simulink model "bengbu_model_DMPC_simple_20260715"  (R2022a)
settings: Solver=VariableStepAuto  StartTime=0.0  StopTime=84700  MaxStep=60  RelTol=1e-3
PreLoadFcn:
  | load('MPC_newmodel_20260715.mat');
InitFcn:
  | load('MPC_newmodel_20260715.mat');
StartFcn:
  | bengbu_0715_reset_workspace; bengbu_0715_export_block_params;
StopFcn:
  | bengbu_0715_schedule_finalize
undefined symbols (not defined in the file or in its folder): case3_startup_trim_prec_state, case3_startup_trim_rec_state, case3_startup_trim_reheat_state, case3_startup_trim_room_state
libraries: slpidlib x3, simulink x3, mpclib x1
settings Model: SimulationMode=accelerator  Creator=73906  LastModifiedBy=73906
settings DataIOCC: SaveOutput=off  SaveTime=off  ReturnWorkspaceOutputs=off

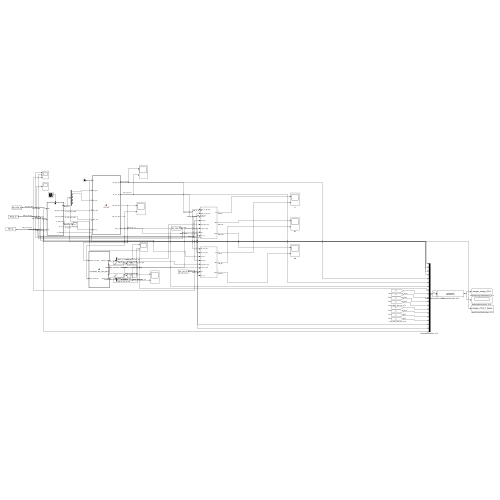
[thumbnail: Simulink's stored preview of the top-level diagram]
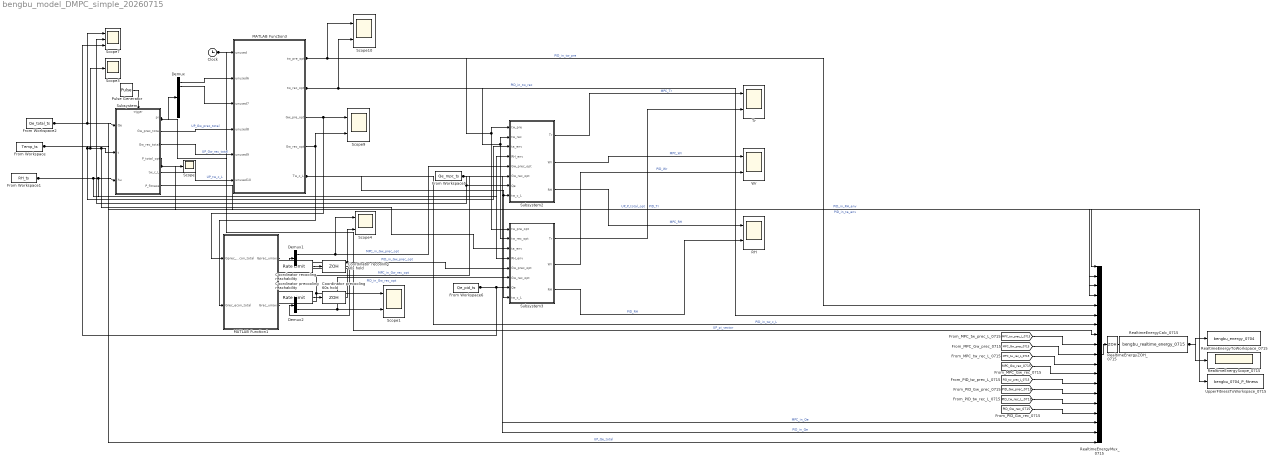
== system bengbu_model_DMPC_simple_20260715 ==
  Clock : Clock
  Coordinator precooling 60s hold : ZeroOrderHold  SampleTime=60
  Coordinator precooling reachability : RateLimiter  RisingSlewLimit=inf  FallingSlewLimit=-0.0116666666666667  InitialCondition=[4.765;4.765]
  Coordinator recooling 60s hold : ZeroOrderHold  SampleTime=60
  Coordinator recooling reachability : RateLimiter  RisingSlewLimit=inf  FallingSlewLimit=-0.02  InitialCondition=[13.2155;13.2155]
  Demux : Demux  Outputs=9
  Demux1 : Demux  Outputs=2
  Demux2 : Demux  Outputs=2
  From Workspace : FromWorkspace  VariableName=Temp_ts
  From Workspace1 : FromWorkspace  VariableName=RH_ts
  From Workspace2 : FromWorkspace  VariableName=Qe_total_ts
  From Workspace5 : FromWorkspace  VariableName=Qe_mpc_ts
  From Workspace6 : FromWorkspace  VariableName=Qe_pid_ts
  MATLAB Function1 : MATLAB Function  TreatAsAtomicUnit=on
  MATLAB Function3 : MATLAB Function  TreatAsAtomicUnit=on  SystemSampleTime=300
  Pulse Generator : DiscretePulseGenerator  PulseType=Time based  Period=3600  PulseWidth=1/360000  PhaseDelay=10
  RH : Scope  NumInputPorts=2
  RealtimeEnergyCalc_0715 : MATLABFcn  MATLABFcn=bengbu_realtime_energy_0715  OutputDimensions=31
  RealtimeEnergyMux_0715 : Mux  Inputs=19
  RealtimeEnergyScope_0715 : Scope
  RealtimeEnergyToWorkspace_0715 : ToWorkspace  VariableName=bengbu_energy_0704  SaveFormat=Timeseries  SampleTime=-1
  RealtimeEnergyZOH_0715 : ZeroOrderHold  SampleTime=300
  Scope : Scope
  Scope{1,4,9..10} (4 alike) : Scope  NumInputPorts=2
  Scope3 : Scope
  Scope7 : Scope  NumInputPorts=3
  Subsystem : Subsystem
  Subsystem2 : Subsystem
  Subsystem3 : Subsystem
  Tr : Scope  NumInputPorts=2
  UpperFitnessToWorkspace_0715 : ToWorkspace  VariableName=bengbu_0704_P_fitness  SaveFormat=Timeseries  SampleTime=-1
  Wr : Scope  NumInputPorts=2
  wires:
  Demux/2 -> MATLAB Function3/3(unused7)
  From Workspace1/1 -> Subsystem2/4(RH_env), Subsystem3/4(RH_env), Subsystem/3(hu), RealtimeEnergyMux_0715/3  "PID_in_RH_env"
  Subsystem/2(Gw_prec_total) -> MATLAB Function3/4(unused8)  "UP_Gw_prec_total"
  Subsystem/3(Gw_rec_total) -> MATLAB Function3/5(unused9)  "UP_Gw_rec_total"
  Pulse Generator/1 -> Subsystem/Trigger
  Demux/1 -> MATLAB Function3/2(unused6)
  Subsystem/1(pi) -> Demux/1, RealtimeEnergyMux_0715/8  "UP_pi_vector"
  Clock/1 -> MATLAB Function3/1(unused), RealtimeEnergyMux_0715/1
  MATLAB Function3/3(Gw_pre_opt) -> MATLAB Function1/1(Gprec_econ_total), Scope9/1
  MATLAB Function3/4(Gw_rec_opt) -> MATLAB Function1/2(Grec_econ_total), Scope9/2
  MATLAB Function3/1(tw_pre_opt) -> Subsystem2/1(tw_pre), Subsystem3/1(tw_pre_opt), Scope10/1, RealtimeEnergyMux_0715/5  "PID_in_tw_pre"
  MATLAB Function3/2(tw_rec_opt) -> Subsystem3/2(tw_rec_opt), Subsystem2/2(tw_rec), Scope10/2, RealtimeEnergyMux_0715/6  "PID_in_tw_rec"
  Subsystem2/1(Tr) -> Tr/1  "MPC_Tr"
  Demux1/1 -> Subsystem2/5(Gw_prec_opt), Scope4/1  "MPC_in_Gw_prec_opt"
  Demux1/2 -> Scope4/2, Subsystem3/5(Gw_prec_opt)  "PID_in_Gw_prec_opt"
  Demux2/1 -> Subsystem2/6(Gw_rec_opt), Scope1/1  "MPC_in_Gw_rec_opt"
  Demux2/2 -> Scope1/2, Subsystem3/6(Gw_rec_opt)  "PID_in_Gw_rec_opt"
  Subsystem3/1(Tr) -> Tr/2  "PID_Tr"
  Subsystem3/2(Wr) -> Wr/2  "PID_Wr"
  Subsystem2/2(Wr) -> Wr/1  "MPC_Wr"
  Subsystem3/3(RH) -> RH/2  "PID_RH"
  From Workspace2/1 -> Scope7/1, Subsystem/1(Qe), RealtimeEnergyMux_0715/19  "UP_Qe_total"
  From Workspace5/1 -> Scope7/2, Subsystem2/7(Qe), RealtimeEnergyMux_0715/17  "MPC_in_Qe"
  Subsystem2/3(RH) -> RH/1  "MPC_RH"
  From Workspace/1 -> Subsystem2/3(ta_env), Scope3/1, Subsystem3/3(ta_env), Subsystem/2(t), RealtimeEnergyMux_0715/2  "PID_in_ta_env"
  From Workspace6/1 -> Scope7/3, Subsystem3/7(Qe), RealtimeEnergyMux_0715/18  "PID_in_Qe"
  Subsystem/5(tw_c_L) -> MATLAB Function3/6(unused10)  "UP_tw_c_L"
  MATLAB Function3/5(Tw_c_L) -> Subsystem2/8(tw_c_L), Subsystem3/8(tw_c_L), RealtimeEnergyMux_0715/7  "PID_in_tw_c_L"
  Subsystem/4(P_total_opt) -> Scope/1, RealtimeEnergyMux_0715/4  "UP_P_total_opt"
  RealtimeEnergyMux_0715/1 -> RealtimeEnergyZOH_0715/1
  RealtimeEnergyCalc_0715/1 -> RealtimeEnergyToWorkspace_0715/1, RealtimeEnergyScope_0715/1
  [MPC_tw_prec_L_0715] -> RealtimeEnergyMux_0715/9
  [MPC_Gw_prec_0715] -> RealtimeEnergyMux_0715/10
  [MPC_tw_rec_L_0715] -> RealtimeEnergyMux_0715/11
  [MPC_Gw_rec_0715] -> RealtimeEnergyMux_0715/12
  [PID_tw_prec_L_0715] -> RealtimeEnergyMux_0715/13
  [PID_Gw_prec_0715] -> RealtimeEnergyMux_0715/14
  [PID_tw_rec_L_0715] -> RealtimeEnergyMux_0715/15
  [PID_Gw_rec_0715] -> RealtimeEnergyMux_0715/16
  RealtimeEnergyZOH_0715/1 -> RealtimeEnergyCalc_0715/1
  Subsystem/6(P_fitness) -> UpperFitnessToWorkspace_0715/1
  MATLAB Function1/1(Gprec_umax) -> Coordinator precooling reachability/1
  Coordinator precooling reachability/1 -> Coordinator precooling 60s hold/1
  Coordinator precooling 60s hold/1 -> Demux1/1
  MATLAB Function1/2(Grec_umax) -> Coordinator recooling reachability/1
  Coordinator recooling reachability/1 -> Coordinator recooling 60s hold/1
  Coordinator recooling 60s hold/1 -> Demux2/1

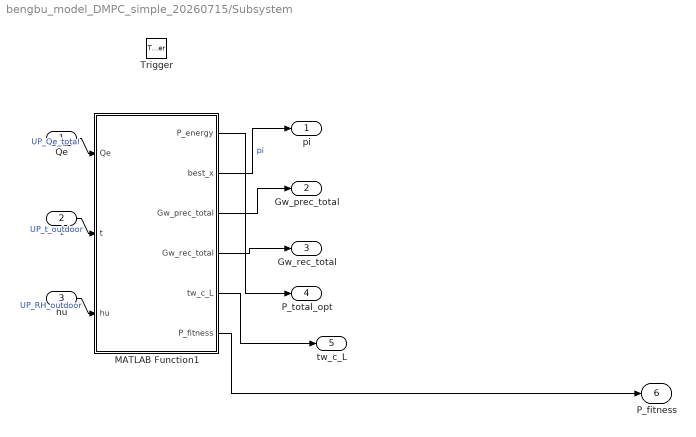
== system bengbu_model_DMPC_simple_20260715/Subsystem ==
  Qe : Inport
  t : Inport  Port=2
  hu : Inport  Port=3
  Trigger : TriggerPort  VariantControl=(inherit)  PortDimensions=1
  MATLAB Function1 : MATLAB Function  TreatAsAtomicUnit=on
  pi : Outport
  Gw_prec_total : Outport  Port=2
  Gw_rec_total : Outport  Port=3
  P_total_opt : Outport  Port=4
  tw_c_L : Outport  Port=5
  P_fitness : Outport  Port=6
  wires:
  MATLAB Function1/4(Gw_rec_total) -> Gw_rec_total/1
  MATLAB Function1/3(Gw_prec_total) -> Gw_prec_total/1
  t/1 -> MATLAB Function1/2(t)  "UP_t_outdoor"
  MATLAB Function1/2(best_x) -> pi/1  "pi"
  hu/1 -> MATLAB Function1/3(hu)  "UP_RH_outdoor"
  Qe/1 -> MATLAB Function1/1(Qe)  "UP_Qe_total"
  MATLAB Function1/1(P_energy) -> P_total_opt/1
  MATLAB Function1/5(tw_c_L) -> tw_c_L/1
  MATLAB Function1/6(P_fitness) -> P_fitness/1

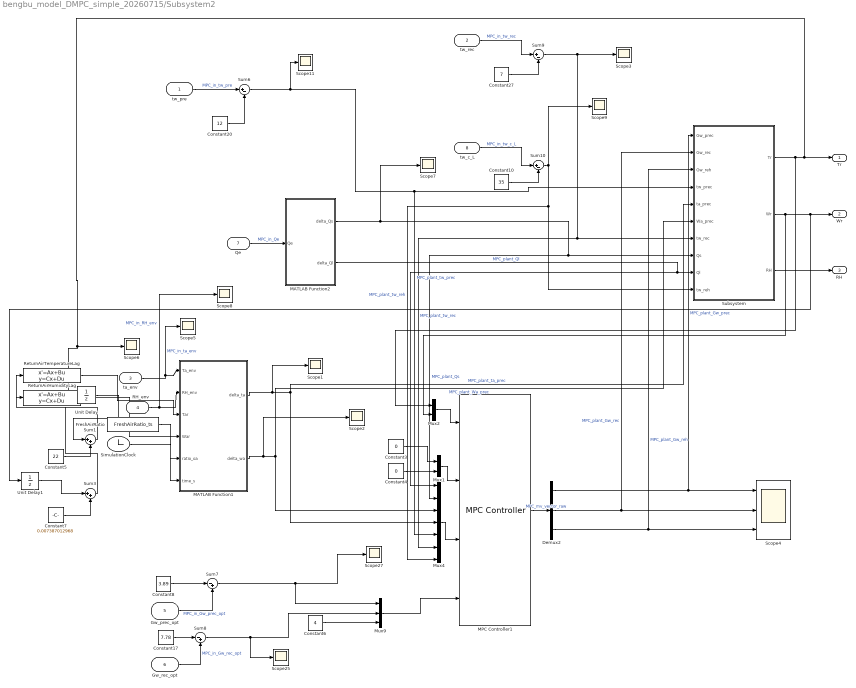
== system bengbu_model_DMPC_simple_20260715/Subsystem2 ==
  tw_pre : Inport
  tw_rec : Inport  Port=2
  ta_env : Inport  Port=3
  RH_env : Inport  Port=4
  Gw_prec_opt : Inport  Port=5
  Gw_rec_opt : Inport  Port=6
  Qe : Inport  Port=7
  tw_c_L : Inport  Port=8
  Constant10 : Constant  Value=35
  Constant17 : Constant  Value=7.78
  Constant20 : Constant  Value=12
  Constant27 : Constant  Value=7
  Constant3 : Constant  Value=0
  Constant4 : Constant  Value=0
  Constant5 : Constant  Value=22
  Constant6 : Constant  Value=4
  Constant7 : Constant  Value=0.007387012968
  Constant8 : Constant  Value=3.89
  Demux2 : Demux  Outputs=3
  FreshAirRatio : FromWorkspace  VariableName=FreshAirRatio_ts
  MATLAB Function1 : MATLAB Function  TreatAsAtomicUnit=on
  MATLAB Function2 : MATLAB Function  TreatAsAtomicUnit=on
  MPC Controller1 : mpclib/MPC Controller  SCDEnableBlockLinearizationSpecification=on  mpcobj=MPC_newmodel_20260704  x0=case3_mpc_initial_state_0715  is_multiple=0  enable_value=0  return_u0=off  updateMPCinCallerWorkspace=off  md_inport=on  mv_inport=off  uref_inport=off  return_cost=off  return_mvseq=off  return_qpstatus=off  return_xseq=off  return_state=off  return_ovseq=off  state_inport=off  umin_inport=off  umax_inport=on  ymin_inport=off  ymax_inport=off  cc_inport=off  ywt_inport=off  uwt_inport=off  duwt_inport=off  rhoeps_inport=off  pm_inport=off  MaximumP=10  HorizonChoice=FixedHorizon  n_ts=60  n_p=60  n_mv=3  n_md=7  n_ud=0  n_mo=2  n_uo=0  BlockDataType=double  SampleTimeInherited=off  switch_inport=off
  Mux1 : Mux  Inputs=2
  Mux2 : Mux  Inputs=2
  Mux4 : Mux  Inputs=7
  Mux9 : Mux  Inputs=3
  ReturnAirHumidityLag : StateSpace  A=-0.00333333333333333  B=0.00333333333333333  D=0  InitialCondition=0.007387012968
  ReturnAirTemperatureLag : StateSpace  A=-0.00333333333333333  B=0.00333333333333333  D=0  InitialCondition=22
  Scope{1..3,5..9,11,25,27} (11 alike) : Scope
  Scope4 : Scope  NumInputPorts=3
  SimulationClock : Clock
  Subsystem : Subsystem
  Sum1 : Sum  Inputs=|++
  Sum10 : Sum  Inputs=|+-
  Sum3 : Sum  Inputs=|++
  Sum6 : Sum  Inputs=|+-
  Sum7 : Sum  Inputs=|-+
  Sum8 : Sum  Inputs=|-+
  Sum9 : Sum  Inputs=|+-
  Unit Delay : UnitDelay  SampleTime=-1  HasFrameUpgradeWarning=on
  Unit Delay1 : UnitDelay  SampleTime=-1  HasFrameUpgradeWarning=on
  Tr : Outport
  Wr : Outport  Port=2
  RH : Outport  Port=3
  wires:
  Sum7/1 -> Scope27/1, Mux9/1
  Constant8/1 -> Sum7/1
  Sum8/1 -> Scope25/1, Mux9/2
  Constant17/1 -> Sum8/1
  Gw_prec_opt/1 -> Sum7/2  "MPC_in_Gw_prec_opt"
  Gw_rec_opt/1 -> Sum8/2  "MPC_in_Gw_rec_opt"
  Sum9/1 -> Mux4/6, Subsystem/7(tw_rec), Scope3/1  "MPC_plant_tw_rec"
  Sum6/1 -> Subsystem/4(tw_prec), Mux4/5, Scope11/1  "MPC_plant_tw_prec"
  Mux4/1 -> MPC Controller1/3
  Mux1/1 -> MPC Controller1/2
  Constant3/1 -> Mux1/1
  Constant4/1 -> Mux1/2
  MPC Controller1/1 -> Demux2/1  "MPC_mv_vector_raw"
  MATLAB Function1/1(delta_ta) -> Scope1/1, Mux4/4, Subsystem/5(ta_prec)  "MPC_plant_ta_prec"
  Constant20/1 -> Sum6/2
  tw_pre/1 -> Sum6/1  "MPC_in_tw_pre"
  Constant27/1 -> Sum9/2
  tw_rec/1 -> Sum9/1  "MPC_in_tw_rec"
  Mux2/1 -> MPC Controller1/1
  Subsystem/1(Tr) -> Unit Delay/1, Scope6/1, Tr/1, Mux2/1
  Subsystem/2(Wr) -> Wr/1, Unit Delay1/1, Mux2/2
  Demux2/1 -> Subsystem/1(Gw_prec), Scope4/1  "MPC_plant_Gw_prec"
  Demux2/2 -> Scope4/2, Subsystem/2(Gw_rec)  "MPC_plant_Gw_rec"
  Demux2/3 -> Subsystem/3(Gw_reh), Scope4/3  "MPC_plant_Gw_reh"
  MATLAB Function1/2(delta_wa) -> Scope2/1, Mux4/3, Subsystem/6(Wa_prec)  "MPC_plant_Wa_prec"
  Qe/1 -> MATLAB Function2/1(Qe)  "MPC_in_Qe"
  MATLAB Function2/1(delta_Qs) -> Scope7/1, Mux4/2, Subsystem/8(Qs)  "MPC_plant_Qs"
  MATLAB Function2/2(delta_Ql) -> Mux4/1, Subsystem/9(Ql)  "MPC_plant_Ql"
  Subsystem/3(RH) -> RH/1
  Constant5/1 -> Sum1/2
  Constant7/1 -> Sum3/2
  Unit Delay/1 -> Sum1/1
  Unit Delay1/1 -> Sum3/1
  ta_env/1 -> Scope5/1, MATLAB Function1/1(Ta_env)  "MPC_in_ta_env"
  RH_env/1 -> Scope8/1, MATLAB Function1/2(RH_env)  "MPC_in_RH_env"
  tw_c_L/1 -> Sum10/1  "MPC_in_tw_c_L"
  Constant10/1 -> Sum10/2
  Sum10/1 -> Scope9/1, Mux4/7, Subsystem/10(tw_reh)  "MPC_plant_tw_reh"
  Mux9/1 -> MPC Controller1/4
  Constant6/1 -> Mux9/3
  FreshAirRatio/1 -> MATLAB Function1/5(ratio_oa)
  SimulationClock/1 -> MATLAB Function1/6(time_s)
  Sum1/1 -> ReturnAirTemperatureLag/1
  ReturnAirTemperatureLag/1 -> MATLAB Function1/3(Tar)
  Sum3/1 -> ReturnAirHumidityLag/1
  ReturnAirHumidityLag/1 -> MATLAB Function1/4(War)

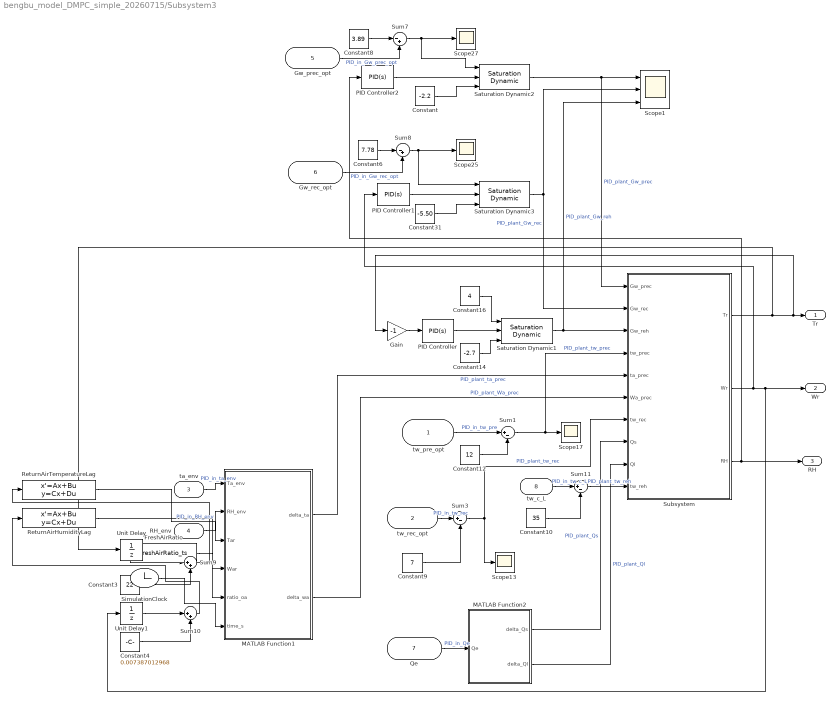
== system bengbu_model_DMPC_simple_20260715/Subsystem3 ==
  tw_pre_opt : Inport
  tw_rec_opt : Inport  Port=2
  ta_env : Inport  Port=3
  RH_env : Inport  Port=4
  Gw_prec_opt : Inport  Port=5
  Gw_rec_opt : Inport  Port=6
  Qe : Inport  Port=7
  tw_c_L : Inport  Port=8
  Constant : Constant  Value=-2.2
  Constant10 : Constant  Value=35
  Constant12 : Constant  Value=12
  Constant14 : Constant  Value=-2.7
  Constant16 : Constant  Value=4
  Constant3 : Constant  Value=22
  Constant31 : Constant  Value=-5.50
  Constant4 : Constant  Value=0.007387012968
  Constant6 : Constant  Value=7.78
  Constant8 : Constant  Value=3.89
  Constant9 : Constant  Value=7
  FreshAirRatio : FromWorkspace  VariableName=FreshAirRatio_ts
  Gain : Gain  Gain=-1
  MATLAB Function1 : MATLAB Function  TreatAsAtomicUnit=on
  MATLAB Function2 : MATLAB Function  TreatAsAtomicUnit=on
  PID Controller : slpidlib/PID Controller  Controller=PID  Form=Ideal  TimeDomain=Continuous-time  UseExternalTs=off  SampleTime=-1  IntegratorMethod=Forward Euler  FilterMethod=Forward Euler  ControllerParametersSource=internal  P=0.52  I=0.0038  UseKiTs=off  D=0.008  N=60  UseFilter=on  TunerSelectOption=Transfer Function Based (PID Tuner App)  InitialConditionSource=internal  InitialConditionForIntegrator=-2.77999999917421  InitialConditionForFilter=0  DifferentiatorICPrevScaledInput=0  ExternalReset=none  TrackingMode=off  Kt=1  LimitOutput=on  SatLimitsSource=internal  UpperSaturationLimit=inf  LowerSaturationLimit=-inf  LinearizeAsGain=on  AntiWindupMode=back-calculation  Kb=1  POutMin=[]  POutMax=[]  IOutMin=[]  IOutMax=[]  DOutMin=[]  DOutMax=[]  NOutMin=[]  NOutMax=[]  SumOutMin=[]  SumOutMax=[]  SaturationOutMin=[]  SaturationOutMax=[]  PParamMin=[]  PParamMax=[]  IParamMin=[]  IParamMax=[]  DParamMin=[]  DParamMax=[]  NParamMin=[]  NParamMax=[]  KbParamMin=[]  KbParamMax=[]  KtParamMin=[]  KtParamMax=[]  KbOutMin=[]  KbOutMax=[]  KtOutMin=[]  KtOutMax=[]  IntegratorOutMin=[]  IntegratorOutMax=[]  FilterOutMin=[]  FilterOutMax=[]  SumI1OutMin=[]  SumI1OutMax=[]  SumI2OutMin=[]  SumI2OutMax=[]  SumI3OutMin=[]  SumI3OutMax=[]  SumI4OutMin=[]  SumI4OutMax=[]  SumDOutMin=[]  SumDOutMax=[]  DifferentiatorOutMin=[]  DifferentiatorOutMax=[]  FilterDiffOutCoefMin=[]  FilterDiffOutCoefMax=[]  ReciprocalOutMin=[]  ReciprocalOutMax=[]  SumDenOutMin=[]  SumDenOutMax=[]  SumNumOutMin=[]  SumNumOutMax=[]  DivideOutMin=[]  DivideOutMax=[]  UdiffTsProdOutMin=[]  UdiffTsProdOutMax=[]  NTsProdOutMin=[]  NTsProdOutMax=[]  UintegralTsProdOutMin=[]  UintegralTsProdOutMax=[]  UngainTsProdOutMin=[]  UngainTsProdOutMax=[]  ClampingZeroOutDataTypeStr=Inherit: Inherit via back propagation  ClampingZeroOutMin=[]  ClampingZeroOutMax=[]  FilterDenConstantOutDataTypeStr=Inherit: Inherit via back propagation  FilterDenConstantOutMin=[]  FilterDenConstantOutMax=[]  PCopyOutDataTypeStr=Inherit: Inherit via back propagation  PCopyOutMin=[]  PCopyOutMax=[]  NCopyOutDataTypeStr=Inherit: Inherit via back propagation  NCopyOutMin=[]  NCopyOutMax=[]  IntegratorContinuousStateAttributes=''  IntegratorStateMustResolveToSignalObject=off  IntegratorRTWStateStorageClass=Auto  FilterContinuousStateAttributes=''  FilterStateMustResolveToSignalObject=off  FilterRTWStateStorageClass=Auto  ParallelPVariant=Passthrough  IdealPVariant=InternalParameters  IVariant=InternalParameters  DVariant=InternalParameters  IntegratorVariant=Continuous  SatVariant=Enabled  AWVariant=BackCalculation  PCopyVariant=Disabled  TRVariant=Disabled  FdbkBlocksVariant=Forward  IdealPFdbkVariant=Disabled  SatFdbkVariant=Disabled  DerivativeFilterVariant=ContFilter  NVariant=InternalParameters  NCopyVariant=Disabled  FilterICVariant=InternalICsFilter  IntegratorICVariant=InternalICs  ExternalResetVariant=Disabled  TRSumVariant=Passthrough  SumFdbkVariant=Disabled  SumVariant=Sum_PID  TsampFilterVariant=InternalTs  TsampNgainVariant=Passthrough  TsampIntegralVariant=Passthrough  ExternalSaturationOutDataTypeStr=Inherit: Same as second input  aMode=0
  PID Controller1 : slpidlib/PID Controller  Controller=PID  Form=Parallel  TimeDomain=Continuous-time  UseExternalTs=off  SampleTime=-1  IntegratorMethod=Forward Euler  FilterMethod=Forward Euler  ControllerParametersSource=internal  P=10000  I=0.65  UseKiTs=off  D=0  N=50  UseFilter=on  TunerSelectOption=Transfer Function Based (PID Tuner App)  InitialConditionSource=internal  InitialConditionForIntegrator=-2.04213946993275  InitialConditionForFilter=0  DifferentiatorICPrevScaledInput=0  ExternalReset=none  TrackingMode=off  Kt=1  LimitOutput=on  SatLimitsSource=internal  UpperSaturationLimit=inf  LowerSaturationLimit=-inf  LinearizeAsGain=on  AntiWindupMode=back-calculation  Kb=1  POutMin=[]  POutMax=[]  IOutMin=[]  IOutMax=[]  DOutMin=[]  DOutMax=[]  NOutMin=[]  NOutMax=[]  SumOutMin=[]  SumOutMax=[]  SaturationOutMin=[]  SaturationOutMax=[]  PParamMin=[]  PParamMax=[]  IParamMin=[]  IParamMax=[]  DParamMin=[]  DParamMax=[]  NParamMin=[]  NParamMax=[]  KbParamMin=[]  KbParamMax=[]  KtParamMin=[]  KtParamMax=[]  KbOutMin=[]  KbOutMax=[]  KtOutMin=[]  KtOutMax=[]  IntegratorOutMin=[]  IntegratorOutMax=[]  FilterOutMin=[]  FilterOutMax=[]  SumI1OutMin=[]  SumI1OutMax=[]  SumI2OutMin=[]  SumI2OutMax=[]  SumI3OutMin=[]  SumI3OutMax=[]  SumI4OutMin=[]  SumI4OutMax=[]  SumDOutMin=[]  SumDOutMax=[]  DifferentiatorOutMin=[]  DifferentiatorOutMax=[]  FilterDiffOutCoefMin=[]  FilterDiffOutCoefMax=[]  ReciprocalOutMin=[]  ReciprocalOutMax=[]  SumDenOutMin=[]  SumDenOutMax=[]  SumNumOutMin=[]  SumNumOutMax=[]  DivideOutMin=[]  DivideOutMax=[]  UdiffTsProdOutMin=[]  UdiffTsProdOutMax=[]  NTsProdOutMin=[]  NTsProdOutMax=[]  UintegralTsProdOutMin=[]  UintegralTsProdOutMax=[]  UngainTsProdOutMin=[]  UngainTsProdOutMax=[]  ClampingZeroOutDataTypeStr=Inherit: Inherit via back propagation  ClampingZeroOutMin=[]  ClampingZeroOutMax=[]  FilterDenConstantOutDataTypeStr=Inherit: Inherit via back propagation  FilterDenConstantOutMin=[]  FilterDenConstantOutMax=[]  PCopyOutDataTypeStr=Inherit: Inherit via back propagation  PCopyOutMin=[]  PCopyOutMax=[]  NCopyOutDataTypeStr=Inherit: Inherit via back propagation  NCopyOutMin=[]  NCopyOutMax=[]  IntegratorContinuousStateAttributes=''  IntegratorStateMustResolveToSignalObject=off  IntegratorRTWStateStorageClass=Auto  FilterContinuousStateAttributes=''  FilterStateMustResolveToSignalObject=off  FilterRTWStateStorageClass=Auto  ParallelPVariant=InternalParameters  IdealPVariant=Disabled  IVariant=InternalParameters  DVariant=InternalParameters  IntegratorVariant=Continuous  SatVariant=Enabled  AWVariant=BackCalculation  PCopyVariant=Disabled  TRVariant=Disabled  FdbkBlocksVariant=Forward  IdealPFdbkVariant=Disabled  SatFdbkVariant=Disabled  DerivativeFilterVariant=ContFilter  NVariant=InternalParameters  NCopyVariant=Disabled  FilterICVariant=InternalICsFilter  IntegratorICVariant=InternalICs  ExternalResetVariant=Disabled  TRSumVariant=Passthrough  SumFdbkVariant=Disabled  SumVariant=Sum_PID  TsampFilterVariant=InternalTs  TsampNgainVariant=Passthrough  TsampIntegralVariant=Passthrough  ExternalSaturationOutDataTypeStr=Inherit: Same as second input  aMode=0
  PID Controller2 : slpidlib/PID Controller  Controller=PID  Form=Parallel  TimeDomain=Continuous-time  UseExternalTs=off  SampleTime=-1  IntegratorMethod=Forward Euler  FilterMethod=Forward Euler  ControllerParametersSource=internal  P=7.2  I=0.005  UseKiTs=off  D=0  N=50  UseFilter=on  TunerSelectOption=Transfer Function Based (PID Tuner App)  InitialConditionSource=internal  InitialConditionForIntegrator=-3.88999999434337  InitialConditionForFilter=0  DifferentiatorICPrevScaledInput=0  ExternalReset=none  TrackingMode=off  Kt=1  LimitOutput=on  SatLimitsSource=internal  UpperSaturationLimit=inf  LowerSaturationLimit=-inf  LinearizeAsGain=on  AntiWindupMode=back-calculation  Kb=1  POutMin=[]  POutMax=[]  IOutMin=[]  IOutMax=[]  DOutMin=[]  DOutMax=[]  NOutMin=[]  NOutMax=[]  SumOutMin=[]  SumOutMax=[]  SaturationOutMin=[]  SaturationOutMax=[]  PParamMin=[]  PParamMax=[]  IParamMin=[]  IParamMax=[]  DParamMin=[]  DParamMax=[]  NParamMin=[]  NParamMax=[]  KbParamMin=[]  KbParamMax=[]  KtParamMin=[]  KtParamMax=[]  KbOutMin=[]  KbOutMax=[]  KtOutMin=[]  KtOutMax=[]  IntegratorOutMin=[]  IntegratorOutMax=[]  FilterOutMin=[]  FilterOutMax=[]  SumI1OutMin=[]  SumI1OutMax=[]  SumI2OutMin=[]  SumI2OutMax=[]  SumI3OutMin=[]  SumI3OutMax=[]  SumI4OutMin=[]  SumI4OutMax=[]  SumDOutMin=[]  SumDOutMax=[]  DifferentiatorOutMin=[]  DifferentiatorOutMax=[]  FilterDiffOutCoefMin=[]  FilterDiffOutCoefMax=[]  ReciprocalOutMin=[]  ReciprocalOutMax=[]  SumDenOutMin=[]  SumDenOutMax=[]  SumNumOutMin=[]  SumNumOutMax=[]  DivideOutMin=[]  DivideOutMax=[]  UdiffTsProdOutMin=[]  UdiffTsProdOutMax=[]  NTsProdOutMin=[]  NTsProdOutMax=[]  UintegralTsProdOutMin=[]  UintegralTsProdOutMax=[]  UngainTsProdOutMin=[]  UngainTsProdOutMax=[]  ClampingZeroOutDataTypeStr=Inherit: Inherit via back propagation  ClampingZeroOutMin=[]  ClampingZeroOutMax=[]  FilterDenConstantOutDataTypeStr=Inherit: Inherit via back propagation  FilterDenConstantOutMin=[]  FilterDenConstantOutMax=[]  PCopyOutDataTypeStr=Inherit: Inherit via back propagation  PCopyOutMin=[]  PCopyOutMax=[]  NCopyOutDataTypeStr=Inherit: Inherit via back propagation  NCopyOutMin=[]  NCopyOutMax=[]  IntegratorContinuousStateAttributes=''  IntegratorStateMustResolveToSignalObject=off  IntegratorRTWStateStorageClass=Auto  FilterContinuousStateAttributes=''  FilterStateMustResolveToSignalObject=off  FilterRTWStateStorageClass=Auto  ParallelPVariant=InternalParameters  IdealPVariant=Disabled  IVariant=InternalParameters  DVariant=InternalParameters  IntegratorVariant=Continuous  SatVariant=Enabled  AWVariant=BackCalculation  PCopyVariant=Disabled  TRVariant=Disabled  FdbkBlocksVariant=Forward  IdealPFdbkVariant=Disabled  SatFdbkVariant=Disabled  DerivativeFilterVariant=ContFilter  NVariant=InternalParameters  NCopyVariant=Disabled  FilterICVariant=InternalICsFilter  IntegratorICVariant=InternalICs  ExternalResetVariant=Disabled  TRSumVariant=Passthrough  SumFdbkVariant=Disabled  SumVariant=Sum_PID  TsampFilterVariant=InternalTs  TsampNgainVariant=Passthrough  TsampIntegralVariant=Passthrough  ExternalSaturationOutDataTypeStr=Inherit: Same as second input  aMode=0
  ReturnAirHumidityLag : StateSpace  A=-0.00333333333333333  B=0.00333333333333333  D=0  InitialCondition=0.007387012968
  ReturnAirTemperatureLag : StateSpace  A=-0.00333333333333333  B=0.00333333333333333  D=0  InitialCondition=22
  Saturation Dynamic1 : simulink/Discontinuities/Saturation Dynamic  OutMin=[]  OutMax=[]  OutDataTypeStr=Inherit: Same as second input  OutDataType=fixdt(1, 16)  OutScaling=2^-10  DoSatur=on
  Saturation Dynamic2 : simulink/Discontinuities/Saturation Dynamic  OutMin=[]  OutMax=[]  OutDataTypeStr=Inherit: Same as second input  OutDataType=fixdt(1, 16)  OutScaling=2^-10  DoSatur=on
  Saturation Dynamic3 : simulink/Discontinuities/Saturation Dynamic  OutMin=[]  OutMax=[]  OutDataTypeStr=Inherit: Same as second input  OutDataType=fixdt(1, 16)  OutScaling=2^-10  DoSatur=on
  Scope1 : Scope  NumInputPorts=3
  Scope{13,17,25,27} (4 alike) : Scope
  SimulationClock : Clock
  Subsystem : Subsystem
  Sum1 : Sum  Inputs=|+-
  Sum10 : Sum  Inputs=|++
  Sum11 : Sum  Inputs=|+-
  Sum3 : Sum  Inputs=|+-
  Sum7 : Sum  Inputs=|-+
  Sum8 : Sum  Inputs=|-+
  Sum9 : Sum  Inputs=|++
  Unit Delay : UnitDelay  SampleTime=-1  HasFrameUpgradeWarning=on
  Unit Delay1 : UnitDelay  SampleTime=-1  HasFrameUpgradeWarning=on
  Tr : Outport
  Wr : Outport  Port=2
  RH : Outport  Port=3
  wires:
  Constant8/1 -> Sum7/1
  Sum3/1 -> Subsystem/7(tw_rec), Scope13/1  "PID_plant_tw_rec"
  Constant6/1 -> Sum8/1
  Gw_prec_opt/1 -> Sum7/2  "PID_in_Gw_prec_opt"
  Gw_rec_opt/1 -> Sum8/2  "PID_in_Gw_rec_opt"
  Gain/1 -> PID Controller/1
  tw_pre_opt/1 -> Sum1/1  "PID_in_tw_pre"
  Constant12/1 -> Sum1/2
  Constant9/1 -> Sum3/2
  tw_rec_opt/1 -> Sum3/1  "PID_in_tw_rec"
  Subsystem/2(Wr) -> PID Controller1/1, Unit Delay1/1, Wr/1
  Sum7/1 -> Saturation Dynamic2/1, Scope27/1
  Sum1/1 -> Subsystem/4(tw_prec), Scope17/1  "PID_plant_tw_prec"
  Qe/1 -> MATLAB Function2/1(Qe)  "PID_in_Qe"
  MATLAB Function2/1(delta_Qs) -> Subsystem/8(Qs)  "PID_plant_Qs"
  MATLAB Function2/2(delta_Ql) -> Subsystem/9(Ql)  "PID_plant_Ql"
  RH_env/1 -> MATLAB Function1/2(RH_env)  "PID_in_RH_env"
  ta_env/1 -> MATLAB Function1/1(Ta_env)  "PID_in_ta_env"
  MATLAB Function1/1(delta_ta) -> Subsystem/5(ta_prec)  "PID_plant_ta_prec"
  MATLAB Function1/2(delta_wa) -> Subsystem/6(Wa_prec)  "PID_plant_Wa_prec"
  Subsystem/3(RH) -> RH/1, PID Controller2/1
  Constant3/1 -> Sum9/2
  Constant4/1 -> Sum10/2
  Unit Delay/1 -> Sum9/1
  Unit Delay1/1 -> Sum10/1
  Sum8/1 -> Scope25/1, Saturation Dynamic3/1
  PID Controller1/1 -> Saturation Dynamic3/2
  PID Controller/1 -> Saturation Dynamic1/2
  Subsystem/1(Tr) -> Unit Delay/1, Tr/1, Gain/1
  Constant14/1 -> Saturation Dynamic1/3
  Constant16/1 -> Saturation Dynamic1/1
  Saturation Dynamic1/1 -> Subsystem/3(Gw_reh), Scope1/3  "PID_plant_Gw_reh"
  Sum11/1 -> Subsystem/10(tw_reh)  "PID_plant_tw_reh"
  Constant10/1 -> Sum11/2
  tw_c_L/1 -> Sum11/1  "PID_in_tw_c_L"
  PID Controller2/1 -> Saturation Dynamic2/2
  Saturation Dynamic3/1 -> Subsystem/2(Gw_rec), Scope1/2  "PID_plant_Gw_rec"
  Saturation Dynamic2/1 -> Scope1/1, Subsystem/1(Gw_prec)  "PID_plant_Gw_prec"
  Constant/1 -> Saturation Dynamic2/3
  Constant31/1 -> Saturation Dynamic3/3
  FreshAirRatio/1 -> MATLAB Function1/5(ratio_oa)
  SimulationClock/1 -> MATLAB Function1/6(time_s)
  Sum9/1 -> ReturnAirTemperatureLag/1
  ReturnAirTemperatureLag/1 -> MATLAB Function1/3(Tar)
  Sum10/1 -> ReturnAirHumidityLag/1
  ReturnAirHumidityLag/1 -> MATLAB Function1/4(War)

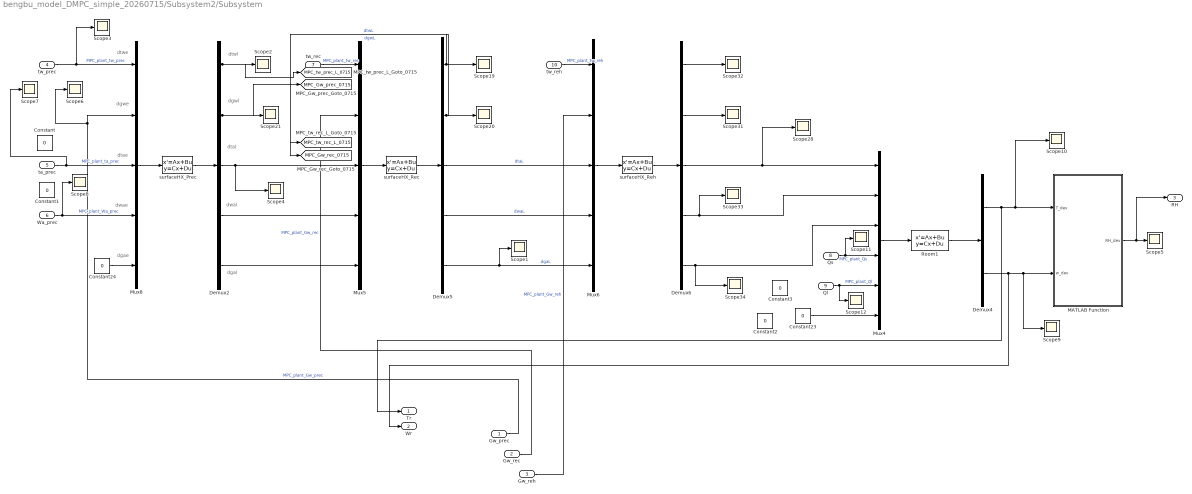
== system bengbu_model_DMPC_simple_20260715/Subsystem2/Subsystem ==
  note: dgal
  note: dwae
  note: dtwl
  note: dgwe
  note: dtwe
  note: dgae
  note: dgwl
  note: dtal
  note: dtae
  note: dwal
  Gw_prec : Inport
  Gw_rec : Inport  Port=2
  Gw_reh : Inport  Port=3
  tw_prec : Inport  Port=4
  ta_prec : Inport  Port=5
  Wa_prec : Inport  Port=6
  tw_rec : Inport  Port=7
  Qs : Inport  Port=8
  Ql : Inport  Port=9
  tw_reh : Inport  Port=10
  Constant{,1..3,23..24} (6 alike) : Constant  Value=0
  Demux2 : Demux  Outputs=5
  Demux4 : Demux  Outputs=2
  Demux5 : Demux  Outputs=5
  Demux6 : Demux  Outputs=5
  MATLAB Function : MATLAB Function  TreatAsAtomicUnit=on
  Mux4 : Mux  Inputs=6
  Mux5 : Mux  Inputs=5
  Mux6 : Mux  Inputs=5
  Mux8 : Mux  Inputs=5
  Room1 : StateSpace  A=[-0.022019 0.000000 0.004809; 0.000000 -0.017210 0.000000; 0.000018 0.000000 -0.000019]  B=[0.01721 0 -0.011852 2e-06 0 0;0 0.01721 -1e-06 0 7.40449874569541e-10 0;0 0 0 0 0 0]  C=[1 0 0;0 1 0]  D=[0 0 0 0 0 0;0 0 0 0 0 0]  InitialCondition=case3_startup_trim_room_state
  Scope{1..12,19..21,28,31..34} (20 alike) : Scope
  surfaceHX_Prec : StateSpace  A=[-0.024378 0.000000 0.000000 0.029414; 0.000000 -3.321515 40.408018 0.656500; 0.000000 -0.000141 -3.673509 0.000658; 0.827965 0.072033 175.283353 -1.895349]  B=[-0.005036 -0.009409 0.000000 0.000000 0.000000; 0.000000 0.000000 2.345190 40.408018 1.586149; 0.000000 0.000000 -0.000141 2.291039 0.000128; 0.827965 -0.681297 0.072033 175.283353 0.202532]  C=[1 0 0 0; 0 0 0 0; 0 1 0 0; 0 0 1 0; 0 0 0 0]  D="[0  0  0  0  0;  0  1  0  0  0;  0  0  0  0  0;  0  0  0  0  0;  0  0  0  0  1]"  InitialCondition=case3_startup_trim_prec_state
  surfaceHX_Rec : StateSpace  A=[-0.022065 0.000000 0.000000 0.021509; 0.000000 -5.290152 83.982152 1.745262; 0.000000 -0.000114 -5.822989 0.001295; 1.035298 0.084317 247.687225 -2.423049]  B=[0.000557 -0.0277425 0 0 0;0 0 3.161221 83.982152 4.257583;0 0 -0.000114 2.949727 0.001017;1.035298 -1.4375835 0.084317 247.687225 0.184959]  C=[1 0 0 0; 0 0 0 0; 0 1 0 0; 0 0 1 0; 0 0 0 0]  D="[0  0  0  0  0;  0  1  0  0  0;  0  0  0  0  0;  0  0  0  0  0;  0  0  0  0  1]"  InitialCondition=case3_startup_trim_rec_state
  surfaceHX_Reh : StateSpace  A=[-0.010968 0.000000 0.014261; 0.000000 -4.978049 4.891414; 1.204247 0.072655 -2.553803]  B=[-0.003293 0.004854 0.000000 0.000000 0.000000; 0.000000 0.000000 3.755195 0.000000 -0.959498; 1.204247 0.346823 0.072655 0.000000 -0.104909]  C="[1  0  0; 0  0  0; 0  1  0;  0  0  0;  0  0  0]"  D="[0  0  0  0  0;  0  1  0  0  0;  0  0  0  0  0;  0  0  0  1  0;  0  0  0  0  1]"  InitialCondition=case3_startup_trim_reheat_state
  Tr : Outport
  Wr : Outport  Port=2
  RH : Outport  Port=3
  tag scope: MPC_Gw_prec_0715=global, MPC_Gw_rec_0715=global, MPC_tw_prec_L_0715=global, MPC_tw_rec_L_0715=global
  wires:
  Demux6/5 -> Mux4/3, Scope34/1
  Demux4/1 -> Tr/1, MATLAB Function/1(T_dev), Scope10/1
  Demux5/1 -> Scope19/1, [MPC_tw_rec_L_0715]  "dtwL"
  Constant23/1 -> Mux4/6
  surfaceHX_Prec/1 -> Demux2/1
  Demux6/2 -> Scope31/1
  Demux5/5 -> Mux6/5, Scope1/1  "dgaL"
  Demux5/3 -> Mux6/3  "dtaL"
  Mux5/1 -> surfaceHX_Rec/1
  Mux8/1 -> surfaceHX_Prec/1
  MATLAB Function/1(RH_dev) -> RH/1, Scope5/1
  Demux4/2 -> Wr/1, Scope9/1, MATLAB Function/2(w_dev)
  surfaceHX_Rec/1 -> Demux5/1
  tw_reh/1 -> Mux6/1  "MPC_plant_tw_reh"
  Demux5/2 -> Scope20/1, [MPC_Gw_rec_0715]  "dgwL"
  Demux6/4 -> Mux4/2, Scope33/1
  Demux6/3 -> Scope28/1, Mux4/1
  Demux2/2 -> Scope21/1, [MPC_Gw_prec_0715]
  Constant24/1 -> Mux8/5
  Demux2/3 -> Mux5/3, Scope4/1
  Demux6/1 -> Scope32/1
  Demux2/5 -> Mux5/5
  Demux5/4 -> Mux6/4  "dwaL"
  Room1/1 -> Demux4/1
  Mux4/1 -> Room1/1
  Gw_prec/1 -> Scope6/1, Mux8/2  "MPC_plant_Gw_prec"
  Gw_reh/1 -> Mux6/2  "MPC_plant_Gw_reh"
  Demux2/1 -> Scope2/1, [MPC_tw_prec_L_0715]
  Gw_rec/1 -> Mux5/2  "MPC_plant_Gw_rec"
  tw_rec/1 -> Mux5/1  "MPC_plant_tw_rec"
  Mux6/1 -> surfaceHX_Reh/1
  tw_prec/1 -> Scope3/1, Mux8/1  "MPC_plant_tw_prec"
  Demux2/4 -> Mux5/4
  surfaceHX_Reh/1 -> Demux6/1
  ta_prec/1 -> Scope7/1, Mux8/3  "MPC_plant_ta_prec"
  Wa_prec/1 -> Scope8/1, Mux8/4  "MPC_plant_Wa_prec"
  Qs/1 -> Scope11/1, Mux4/4  "MPC_plant_Qs"
  Ql/1 -> Scope12/1, Mux4/5  "MPC_plant_Ql"

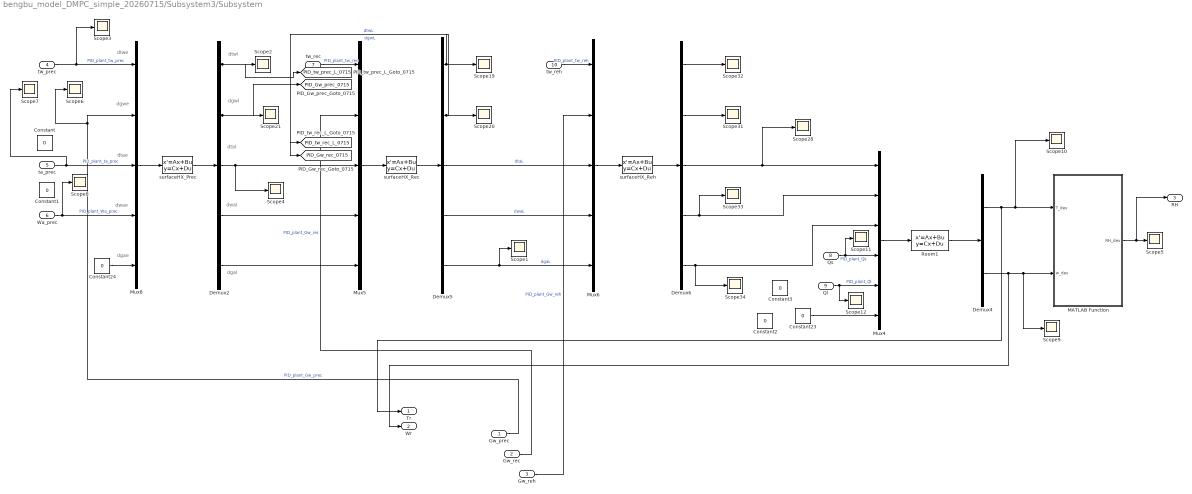
== system bengbu_model_DMPC_simple_20260715/Subsystem3/Subsystem ==
  note: dgal
  note: dwae
  note: dtwl
  note: dgwe
  note: dtwe
  note: dgae
  note: dgwl
  note: dtal
  note: dtae
  note: dwal
  Gw_prec : Inport
  Gw_rec : Inport  Port=2
  Gw_reh : Inport  Port=3
  tw_prec : Inport  Port=4
  ta_prec : Inport  Port=5
  Wa_prec : Inport  Port=6
  tw_rec : Inport  Port=7
  Qs : Inport  Port=8
  Ql : Inport  Port=9
  tw_reh : Inport  Port=10
  Constant{,1..3,23..24} (6 alike) : Constant  Value=0
  Demux2 : Demux  Outputs=5
  Demux4 : Demux  Outputs=2
  Demux5 : Demux  Outputs=5
  Demux6 : Demux  Outputs=5
  MATLAB Function : MATLAB Function  TreatAsAtomicUnit=on
  Mux4 : Mux  Inputs=6
  Mux5 : Mux  Inputs=5
  Mux6 : Mux  Inputs=5
  Mux8 : Mux  Inputs=5
  Room1 : StateSpace  A=[-0.022019 0.000000 0.004809; 0.000000 -0.017210 0.000000; 0.000018 0.000000 -0.000019]  B=[0.01721 0 -0.011852 2e-06 0 0;0 0.01721 -1e-06 0 7.40449874569541e-10 0;0 0 0 0 0 0]  C=[1 0 0;0 1 0]  D=[0 0 0 0 0 0;0 0 0 0 0 0]  InitialCondition=case3_startup_trim_room_state
  Scope{1..12,19..21,28,31..34} (20 alike) : Scope
  surfaceHX_Prec : StateSpace  A=[-0.024378 0.000000 0.000000 0.029414; 0.000000 -3.321515 40.408018 0.656500; 0.000000 -0.000141 -3.673509 0.000658; 0.827965 0.072033 175.283353 -1.895349]  B=[-0.005036 -0.009409 0.000000 0.000000 0.000000; 0.000000 0.000000 2.345190 40.408018 1.586149; 0.000000 0.000000 -0.000141 2.291039 0.000128; 0.827965 -0.681297 0.072033 175.283353 0.202532]  C=[1 0 0 0; 0 0 0 0; 0 1 0 0; 0 0 1 0; 0 0 0 0]  D="[0  0  0  0  0;  0  1  0  0  0;  0  0  0  0  0;  0  0  0  0  0;  0  0  0  0  1]"  InitialCondition=case3_startup_trim_prec_state
  surfaceHX_Rec : StateSpace  A=[-0.022065 0.000000 0.000000 0.021509; 0.000000 -5.290152 83.982152 1.745262; 0.000000 -0.000114 -5.822989 0.001295; 1.035298 0.084317 247.687225 -2.423049]  B=[0.000557 -0.0277425 0 0 0;0 0 3.161221 83.982152 4.257583;0 0 -0.000114 2.949727 0.001017;1.035298 -1.4375835 0.084317 247.687225 0.184959]  C=[1 0 0 0; 0 0 0 0; 0 1 0 0; 0 0 1 0; 0 0 0 0]  D="[0  0  0  0  0;  0  1  0  0  0;  0  0  0  0  0;  0  0  0  0  0;  0  0  0  0  1]"  InitialCondition=case3_startup_trim_rec_state
  surfaceHX_Reh : StateSpace  A=[-0.010968 0.000000 0.014261; 0.000000 -4.978049 4.891414; 1.204247 0.072655 -2.553803]  B=[-0.003293 0.004854 0.000000 0.000000 0.000000; 0.000000 0.000000 3.755195 0.000000 -0.959498; 1.204247 0.346823 0.072655 0.000000 -0.104909]  C="[1  0  0; 0  0  0; 0  1  0;  0  0  0;  0  0  0]"  D="[0  0  0  0  0;  0  1  0  0  0;  0  0  0  0  0;  0  0  0  1  0;  0  0  0  0  1]"  InitialCondition=case3_startup_trim_reheat_state
  Tr : Outport
  Wr : Outport  Port=2
  RH : Outport  Port=3
  tag scope: PID_Gw_prec_0715=global, PID_Gw_rec_0715=global, PID_tw_prec_L_0715=global, PID_tw_rec_L_0715=global
  wires:
  Demux6/5 -> Mux4/3, Scope34/1
  Demux4/1 -> Tr/1, MATLAB Function/1(T_dev), Scope10/1
  Demux5/1 -> Scope19/1, [PID_tw_rec_L_0715]  "dtwL"
  Constant23/1 -> Mux4/6
  surfaceHX_Prec/1 -> Demux2/1
  Demux6/2 -> Scope31/1
  Demux5/5 -> Mux6/5, Scope1/1  "dgaL"
  Demux5/3 -> Mux6/3  "dtaL"
  Mux5/1 -> surfaceHX_Rec/1
  Mux8/1 -> surfaceHX_Prec/1
  MATLAB Function/1(RH_dev) -> RH/1, Scope5/1
  Demux4/2 -> Wr/1, Scope9/1, MATLAB Function/2(w_dev)
  surfaceHX_Rec/1 -> Demux5/1
  tw_reh/1 -> Mux6/1  "PID_plant_tw_reh"
  Demux5/2 -> Scope20/1, [PID_Gw_rec_0715]  "dgwL"
  Demux6/4 -> Mux4/2, Scope33/1
  Demux6/3 -> Scope28/1, Mux4/1
  Demux2/2 -> Scope21/1, [PID_Gw_prec_0715]
  Constant24/1 -> Mux8/5
  Demux2/3 -> Mux5/3, Scope4/1
  Demux6/1 -> Scope32/1
  Demux2/5 -> Mux5/5
  Demux5/4 -> Mux6/4  "dwaL"
  Room1/1 -> Demux4/1
  Mux4/1 -> Room1/1
  Gw_prec/1 -> Scope6/1, Mux8/2  "PID_plant_Gw_prec"
  Gw_reh/1 -> Mux6/2  "PID_plant_Gw_reh"
  Demux2/1 -> Scope2/1, [PID_tw_prec_L_0715]
  Gw_rec/1 -> Mux5/2  "PID_plant_Gw_rec"
  tw_rec/1 -> Mux5/1  "PID_plant_tw_rec"
  Mux6/1 -> surfaceHX_Reh/1
  tw_prec/1 -> Scope3/1, Mux8/1  "PID_plant_tw_prec"
  Demux2/4 -> Mux5/4
  surfaceHX_Reh/1 -> Demux6/1
  ta_prec/1 -> Scope7/1, Mux8/3  "PID_plant_ta_prec"
  Wa_prec/1 -> Scope8/1, Mux8/4  "PID_plant_Wa_prec"
  Qs/1 -> Scope11/1, Mux4/4  "PID_plant_Qs"
  Ql/1 -> Scope12/1, Mux4/5  "PID_plant_Ql"

== matlab function bengbu_model_DMPC_simple_20260715/Subsystem2/MATLAB Function1 ==
  data: Ta_env input; delta_ta output; RH_env input; Tar input; War input; delta_wa output; ratio_oa input; time_s input
function [delta_ta, delta_wa] = calc_air(Ta_env, RH_env, Tar, War, ratio_oa, time_s)
% 使用统一的平滑新风比时间序列，再计算物理混风状态。
P = 101325;
ta0 = 26;
wa0 = 0.0116;
[Ta_mix,Wa_mix] = case3_mixed_air_state_0715( ...
    Ta_env,RH_env,Tar,War,ratio_oa,P);
delta_ta = Ta_mix - ta0;
delta_wa = Wa_mix - wa0;
% 混风状态从首个采样点起直接采用calc_air实时物理计算值。
end

== matlab function bengbu_model_DMPC_simple_20260715/Subsystem2/MATLAB Function2 ==
  data: Qe input; delta_Qs output; delta_Ql output
function [delta_Qs, delta_Ql] = calc_coolingload(Qe)
% Qe is the cooling load of one representative 40-AHU branch, kW.
N_AHU_branch = 40;
Qe_each = Qe / N_AHU_branch;
Qs0 = 60 * 1000;
Ql0 = 15 * 1000;
SHR = 0.85;
Qs = SHR * Qe_each * 1000;
Ql = (1-SHR) * Qe_each * 1000;
delta_Qs = Qs - Qs0;
delta_Ql = Ql - Ql0;
end

== matlab function bengbu_model_DMPC_simple_20260715/Subsystem3/MATLAB Function1 ==
  data: Ta_env input; delta_ta output; RH_env input; Tar input; War input; delta_wa output; ratio_oa input; time_s input
function [delta_ta, delta_wa] = calc_air(Ta_env, RH_env, Tar, War, ratio_oa, time_s)
% 使用统一的平滑新风比时间序列，再计算物理混风状态。
P = 101325;
ta0 = 26;
wa0 = 0.0116;
[Ta_mix,Wa_mix] = case3_mixed_air_state_0715( ...
    Ta_env,RH_env,Tar,War,ratio_oa,P);
delta_ta = Ta_mix - ta0;
delta_wa = Wa_mix - wa0;
% 混风状态从首个采样点起直接采用calc_air实时物理计算值。
end

== matlab function bengbu_model_DMPC_simple_20260715/Subsystem/MATLAB Function1 ==
  data: P_energy output; Qe input; best_x output; t input; hu input; Gw_prec_total output; Gw_rec_total output; tw_c_L output; P_fitness output
function [P_energy,best_x, Gw_prec_total, Gw_rec_total, tw_c_L, P_fitness] = TIEO_Controller(Qe, t, hu)
%#codegen

coder.extrinsic('TIEO_run_wrapper_reheat_0715');

best_x = zeros(1,9);
Gw_prec_total = 0.0;
Gw_rec_total  = 0.0;
P_energy = 0.0;
P_fitness = 0.0;
tw_c_L = 0.0;

best_x_tmp = zeros(1,9);
Gw_prec_tmp = 0.0;
Gw_rec_tmp  = 0.0;
P_energy_tmp = 0.0;
P_fitness_tmp = 0.0;
Tw_tmp = 0.0;

[P_fitness_tmp, P_energy_tmp, best_x_tmp, Gw_prec_tmp, Gw_rec_tmp, Tw_tmp] = ...
    TIEO_run_wrapper_reheat_0715(double(Qe), double(t), double(hu));

best_x = reshape(double(best_x_tmp), 1, 9);
Gw_prec_total = double(Gw_prec_tmp);
Gw_rec_total  = double(Gw_rec_tmp);
P_energy = double(P_energy_tmp);
P_fitness = double(P_fitness_tmp);
tw_c_L = double(Tw_tmp);

end

== matlab function bengbu_model_DMPC_simple_20260715/Subsystem2/Subsystem/MATLAB Function ==
  data: T_dev input; RH_dev output; w_dev input
function RH_dev = calc_RH_dev(T_dev, w_dev)
% 输入：
% T_dev: 温度偏差 ΔT [°C]
% w_dev: 含湿量偏差 Δw [kg/kg]
%
% 输出：
% RH_dev: 相对湿度偏差 ΔRH (相对于 0.45)

%% ===== 基准点 =====
T0 = 22;        % °C
RH0 = 0.45;     % 45%

P = 101325;     % Pa

% 由 T0 和 RH0 反算基准含湿量
Psat0 = 611.2 * exp(17.62 * T0 / (243.12 + T0));
Pv0 = RH0 * Psat0;
w0 = 0.6219 * Pv0 / (P - Pv0);

%% ===== 还原真实状态 =====
T = T0 + T_dev;
w = w0 + w_dev;

%% ===== 饱和蒸汽压 =====
Psat = 611.2 * exp(17.62 * T ./ (243.12 + T));

%% ===== 实际水蒸气分压力 =====
Pv = P * w ./ (0.6219 + w);

%% ===== 相对湿度 =====
RH = Pv ./ Psat;

%% ===== 限幅（物理合理性）=====
RH = min(max(RH, 0), 1);

%% ===== 输出偏差 =====
RH_dev = RH - RH0;

end

== matlab function bengbu_model_DMPC_simple_20260715/MATLAB Function1 ==
  data: Gprec_econ_total input; Grec_econ_total input; Gprec_umax output; Grec_umax output
function [Gprec_umax, Grec_umax] = coordinator_two_zone_0617(Gprec_econ_total, Grec_econ_total)
%#codegen
N_AHU_total = 80;
Gprec_econ_each = max(double(Gprec_econ_total),0) / N_AHU_total;
Grec_econ_each = max(double(Grec_econ_total),0) / N_AHU_total;
Gprec_nom = 3.89; Grec_nom = 7.78;
dGprec_min = -2.5; dGprec_max = 2.5;
dGrec_min = -5.5; dGrec_max = 5.5;
Gprec_reserve = 2.5; Grec_reserve = 3;
Gprec_limit = min(max(Gprec_econ_each+Gprec_reserve,Gprec_nom+dGprec_min),Gprec_nom+dGprec_max);
Grec_limit = min(max(Grec_econ_each+Grec_reserve,Grec_nom+dGrec_min),Grec_nom+dGrec_max);
Gprec_umax = [Gprec_limit;Gprec_limit];
Grec_umax = [Grec_limit;Grec_limit];
end

== matlab function bengbu_model_DMPC_simple_20260715/Subsystem3/MATLAB Function2 ==
  data: Qe input; delta_Qs output; delta_Ql output
function [delta_Qs, delta_Ql] = calc_coolingload(Qe)
% Qe is the cooling load of one representative 40-AHU branch, kW.
N_AHU_branch = 40;
Qe_each = Qe / N_AHU_branch;
Qs0 = 60 * 1000;
Ql0 = 15 * 1000;
SHR = 0.85;
Qs = SHR * Qe_each * 1000;
Ql = (1-SHR) * Qe_each * 1000;
delta_Qs = Qs - Qs0;
delta_Ql = Ql - Ql0;
end

== matlab function bengbu_model_DMPC_simple_20260715/MATLAB Function3 ==
  data: unused input; tw_pre_opt output; unused6 input; unused7 input; unused8 input; unused9 input; tw_rec_opt output; Gw_pre_opt output; Gw_rec_opt output; unused10 input; Tw_c_L output
function [tw_pre_opt,tw_rec_opt,Gw_pre_opt,Gw_rec_opt,Tw_c_L] = init_hold(~,~,~,~,~,~)
%#codegen
tw_pre_opt = 12;
tw_rec_opt = 7;
Gw_pre_opt = 311.2;
Gw_rec_opt = 622.4;
Tw_c_L = 35;
end

== matlab function bengbu_model_DMPC_simple_20260715/Subsystem3/Subsystem/MATLAB Function ==
  data: T_dev input; RH_dev output; w_dev input
function RH_dev = calc_RH_dev(T_dev, w_dev)
% 输入：
% T_dev: 温度偏差 ΔT [°C]
% w_dev: 含湿量偏差 Δw [kg/kg]
%
% 输出：
% RH_dev: 相对湿度偏差 ΔRH (相对于 0.45)

%% ===== 基准点 =====
T0 = 22;        % °C
RH0 = 0.45;     % 45%

P = 101325;     % Pa

% 由 T0 和 RH0 反算基准含湿量
Psat0 = 611.2 * exp(17.62 * T0 / (243.12 + T0));
Pv0 = RH0 * Psat0;
w0 = 0.6219 * Pv0 / (P - Pv0);

%% ===== 还原真实状态 =====
T = T0 + T_dev;
w = w0 + w_dev;

%% ===== 饱和蒸汽压 =====
Psat = 611.2 * exp(17.62 * T ./ (243.12 + T));

%% ===== 实际水蒸气分压力 =====
Pv = P * w ./ (0.6219 + w);

%% ===== 相对湿度 =====
RH = Pv ./ Psat;

%% ===== 限幅（物理合理性）=====
RH = min(max(RH, 0), 1);

%% ===== 输出偏差 =====
RH_dev = RH - RH0;

end
